simulink model "simulink_base_"  (R2014a)
settings: Solver=FixedStepDiscrete  StartTime=0.0  StopTime=500  FixedStep=0.2  RelTol=1e-3
PostLoadFcn:
  | addpath(fileparts(fileparts(get_param(bdroot,'FileName'))),'-begin');
  | configurar_pastas_simulink;
InitFcn:
  | addpath(fileparts(fileparts(get_param(bdroot,'FileName'))),'-begin');
  | configurar_pastas_simulink;
  | % Planta identificada no MATLAB
  | Ts = 0.2;
  | 
  | K = [ ...
  |     0.25190663807022357 ...
  |     3.4791260046895944 ...
  |     20.647834746496613];
  | 
  | tau = [ ...
  |     1.1799856214252014 ...
  |     28.455420541284408 ...
  |     821.62865228021508];
  | 
  | L = 0.5071198600939989; % atraso identificado, em segundos
  | 
  | % Separacao do atraso em parte inteira e fracionaria
  | n_atraso = floor(L / Ts);
  | fracao = L - n_atraso * Ts;
  | 
  | % Discretizacao exata nos instantes de amostragem,
  | % considerando entrada constante entre amostras (ZOH)
  | a = exp(-Ts ./ tau);
  | 
  | b_novo = K .* (-expm1(-(Ts - fracao) ./ tau));
  | 
  | b_anterior = K .* exp(-(Ts - fracao) ./ tau) ...
  |                .* (-expm1(-fracao ./ tau));
  | 
  | % Soma dos tres ramos, incluindo todo o atraso
  | num_planta = zeros(1,4);
  | 
  | for i = 1:3
  |     outros = a;
  |     outros(i) = [];
  | 
  |     num_planta = num_planta + ...
  |         conv([b_novo(i) b_anterior(i)], poly(outros));
  | end
  | 
  | den_planta = [poly(a) zeros(1,n_atraso + 1)];
StartFcn:
  | iniciar_registro_simulacao(bdroot);
StopFcn:
  | exportar_simulacao_comparacao(bdroot);
settings Model: Creator=Thiago  LastModifiedBy=Thiago
settings OptimizationCC: InlineParams=on  OptimizeModelRefInitCode=on  LifeSpan=1
settings HardwareCC: ProdBitPerInt=16  ProdBitPerPointer=8  ProdIntDivRoundTo=Zero  ProdEndianess=LittleEndian  ProdWordSize=8  ProdHWDeviceType=Atmel->AVR
settings RTWCC: SystemTargetFile=ert.tlc  TemplateMakefile=ert_default_tmf  Description=Embedded Coder  ProcessScript=ert_make_rtw_hook
settings CodeAppCC: IgnoreCustomStorageClasses=off
settings ERTTargetCC: GenerateSampleERTMain=off  ParMdlRefBuildCompliant=on  CompOptLevelCompliant=on  ConcurrentExecutionCompliant=on  ERTFirstTimeCompliant=on  SupportNonFinite=off  ModelStepFunctionPrototypeControlCompliant=on  CPPClassGenCompliant=on  InlinedParameterPlacement=Hierarchical  ERTCustomFileTemplate=example_file_process.tlc

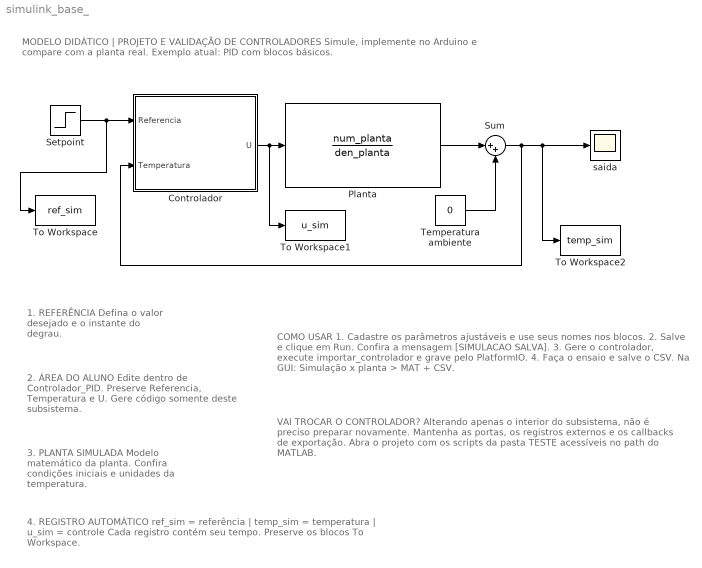
== system simulink_base_ ==
  note: MODELO DIDÁTICO | PROJETO E VALIDAÇÃO DE CONTROLADORES
      | Simule, implemente no Arduino e compare com a planta real.
      | Exemplo atual: PID com blocos básicos.
  note: 1. REFERÊNCIA
      | Defina o valor desejado
      | e o instante do degrau.
  note: 2. ÁREA DO ALUNO
      | Edite dentro de Controlador_PID.
      | Preserve Referencia, Temperatura e U.
      | Gere código somente deste subsistema.
  note: 3. PLANTA SIMULADA
      | Modelo matemático da planta.
      | Confira condições iniciais
      | e unidades da temperatura.
  note: 4. REGISTRO AUTOMÁTICO
      | ref_sim = referência | temp_sim = temperatura | u_sim = controle
      | Cada registro contém seu tempo. Preserve os blocos To Workspace.
  note: COMO USAR
      | 1. Cadastre os parâmetros ajustáveis e use seus nomes nos blocos.
      | 2. Salve e clique em Run. Confira a mensagem [SIMULACAO SALVA].
      | 3. Gere o controlador, execute importar_controlador e grave pelo PlatformIO.
      | 4. Faça o ensaio e salve o CSV. Na GUI: Simulação x planta > MAT + CSV.
  note: VAI TROCAR O CONTROLADOR?
      | Alterando apenas o interior do subsistema, não é preciso preparar novamente.
      | Mantenha as portas, os registros externos e os callbacks de exportação.
      | Abra o projeto com os scripts da pasta TESTE acessíveis no path do MATLAB.
  "Controlador " : Subsystem
  Planta : DiscreteTransferFcn  Numerator=num_planta  Denominator=den_planta  SampleTime=Ts
  Setpoint : Step  Time=0  After=30  SampleTime=0
  Sum : Sum  Inputs=|++
  Temperatura ambiente : Constant  Value=0  VectorParams1D=off
  To Workspace : ToWorkspace  VariableName=ref_sim  SaveFormat=Structure With Time  SampleTime=0.2
  To Workspace1 : ToWorkspace  VariableName=u_sim  SaveFormat=Structure With Time  SampleTime=0.2
  To Workspace2 : ToWorkspace  VariableName=temp_sim  SaveFormat=Structure With Time  SampleTime=0.2
  saida : Scope
  wires:
  "Controlador "/1(U) -> Planta/1, To Workspace1/1
  Setpoint/1 -> "Controlador "/1(Referencia), To Workspace/1
  Planta/1 -> Sum/1
  Temperatura ambiente/1 -> Sum/2
  Sum/1 -> "Controlador "/2(Temperatura), To Workspace2/1, saida/1

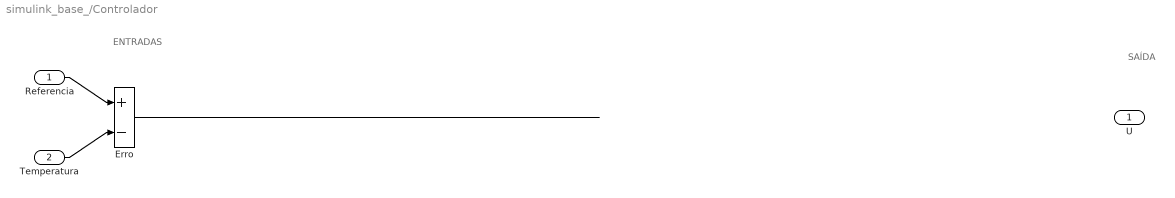
== system simulink_base_/Controlador  ==
  note: SAÍDA
  note: ENTRADAS
  Referencia : Inport
  Temperatura : Inport  Port=2
  Erro : Sum  Inputs=+-  SaturateOnIntegerOverflow=on  InputSameDT=on  OutDataTypeStr=Inherit: Same as first input
  U : Outport
  wires:
  Referencia/1 -> Erro/1
  Temperatura/1 -> Erro/2
  Erro/1 -> ?
  ? -> U/1
